simulink model "autocodeModel"  (R2026a)
settings: Solver=FixedStepDiscrete
settings Model: DataDictionary=navParams.sldd  Creator=maxhu  LastModifiedBy=Christian
settings OptimizationCC: UseDivisionForNetSlopeComputation=on  GainParamInheritBuiltInType=on  UseFloatMulNetSlope=on  InlineInvariantSignals=on  NoFixptDivByZeroProtection=on  EfficientFloat2IntCast=on  LifeSpan=1
settings HardwareCC: ProdLargestAtomicInteger=Long  ProdLargestAtomicFloat=Double  ProdHWDeviceType=ARM Compatible->ARM Cortex-M7 (MPS2)
settings RTWCC: SystemTargetFile=ert.tlc  GenCodeOnly=on  Toolchain=GNU Tools for STM32  BuildConfiguration=Faster Runs  Description=Embedded Coder
settings CodeAppCC: CustomSymbolStrGlobalVar=rt$N$M  CustomSymbolStrType=$N$M  CustomSymbolStrFcn=$N$M$F  CustomSymbolStrMacro=$R_$N$M
settings ERTTargetCC: ERTFilePackagingFormat=CompactWithDataFile  UtilityFuncGeneration=Shared location  GenerateSampleERTMain=on  IncludeMdlTerminateFcn=off  CombineSignalStateStructs=on  SupportAbsoluteTime=off  CodeInterfacePackaging=Reusable function  SupportComplex=off  SupportNonInlinedSFcns=on

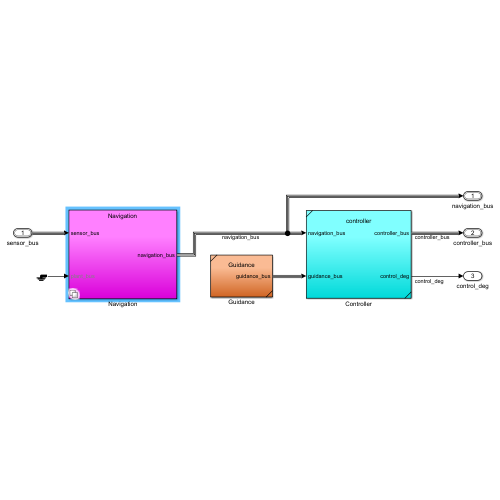
[thumbnail: Simulink's stored preview of the top-level diagram]
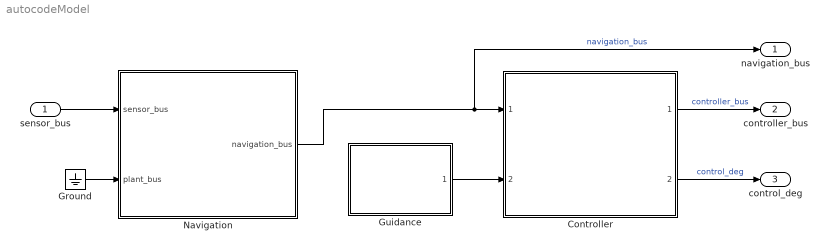
== system autocodeModel ==
  sensor_bus : Inport  OutDataTypeStr=Bus: sensor_bus
  Controller : Subsystem  ReferencedSubsystem=controller
      settings: PermitHierarchicalResolution=None
  Ground : Ground
  Guidance : Subsystem  ReferencedSubsystem=Guidance
      settings: PermitHierarchicalResolution=None
  Navigation : Subsystem  Variant=on
  navigation_bus : Outport  OutDataTypeStr=Bus: navigation_bus
  controller_bus : Outport  Port=2  OutDataTypeStr=Bus: controller_bus
  control_deg : Outport  Port=3
  wires:
  sensor_bus/1 -> Navigation/1(sensor_bus)
  Navigation/1(navigation_bus) -> navigation_bus/1, Controller/1  "navigation_bus"
  Guidance/1 -> Controller/2
  Controller/1 -> controller_bus/1  "controller_bus"
  Ground/1 -> Navigation/2(plant_bus)
  Controller/2 -> control_deg/1  "control_deg"

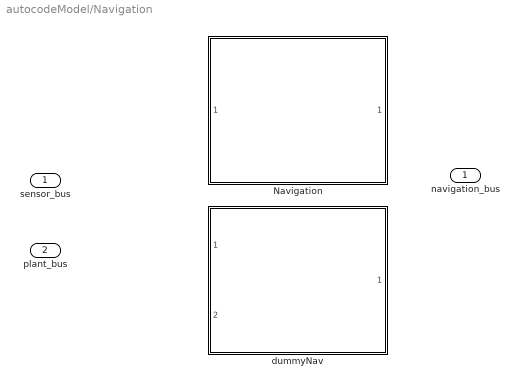
== system autocodeModel/Navigation ==
  sensor_bus : Inport
  plant_bus : Inport  Port=2
  Navigation : Subsystem  VariantControl=navControl.useNav_b == true  ReferencedSubsystem=navigation
      settings: PermitHierarchicalResolution=None
  dummyNav : Subsystem  VariantControl=navControl.useNav_b == false  ReferencedSubsystem=dummyNav
  navigation_bus : Outport
